simulink model "DiscretePIDTest"  (R2026b)
settings: Solver=FixedStepDiscrete  StopTime=pidTestCfg.Duration  FixedStep=pidCfg.Ts
PostLoadFcn:
  | addpath(fullfile(fileparts(get_param('DiscretePIDTest','FileName')),'..','build_process')); initialize_discrete_pid_test('DiscretePIDTest');
model workspace (MAT data in the model file):
  pidCfg.Kp = 1.2
  pidCfg.Ki = 8
  pidCfg.Kd = 0
  pidCfg.Tf = 0.01
  pidCfg.Ts = 0.001
  pidCfg.UMin = -1
  pidCfg.UMax = 1
  pidCfg.X0 = 0
  pidCfg.Kaw = 20
  pidCfg.PlantTau = 0.08
  pidCfg.ClosedLoop = 1
  pidStim.command.time = []
  pidStim.command.signals.values = [0 0 0 0 0 0 0 0 0 0 0 0 ... (3001 elements, 3001x1)]
  pidStim.command.signals.dimensions = 1
  pidStim.enable.time = []
  pidStim.enable.signals.values = [1 1 1 1 1 1 1 1 1 1 1 1 ... (3001 elements, 3001x1)]
  pidStim.enable.signals.dimensions = 1
  pidStim.reset.time = []
  pidStim.reset.signals.values = [0 0 0 0 0 0 0 0 0 0 0 0 ... (3001 elements, 3001x1)]
  pidStim.reset.signals.dimensions = 1
  pidTestCfg.Duration = 3
  pidTestCfg.CommandInitial = 0
  pidTestCfg.CommandHigh = 2
  pidTestCfg.CommandFinal = 0.2
  pidTestCfg.CommandTime = 0.1
  pidTestCfg.ReleaseTime = 1
  pidTestCfg.Enable = 1
  pidTestCfg.Reset = 0
libraries: slpidlib x1, DiscretePID x1
settings Model: Creator=24322  LastModifiedBy=24322
settings DataIOCC: SignalLogging=off

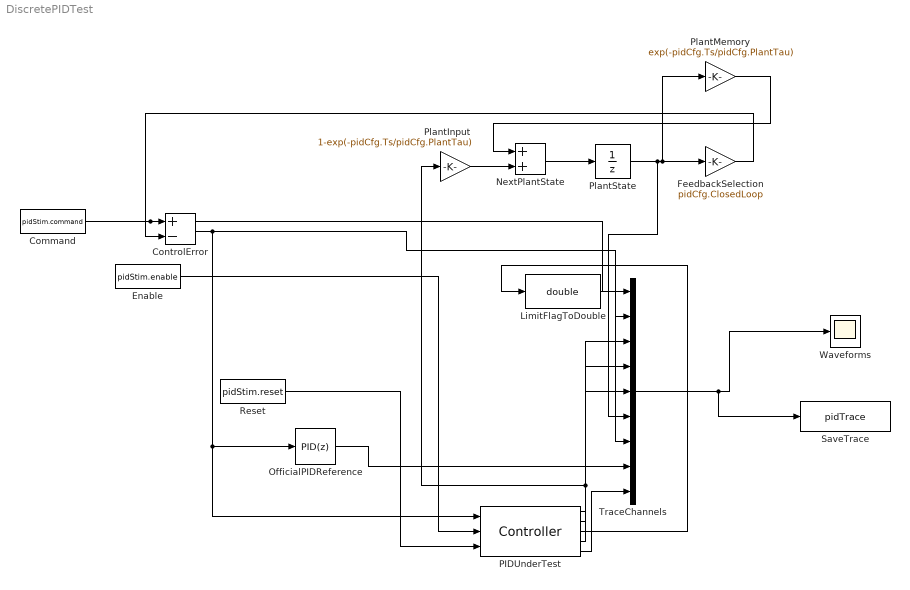
== system DiscretePIDTest ==
  Command : FromWorkspace  VariableName=pidStim.command  SampleTime=pidCfg.Ts  Interpolate=off  OutputAfterFinalValue=Holding final value
  ControlError : Sum  Inputs=+-
  Enable : FromWorkspace  VariableName=pidStim.enable  SampleTime=pidCfg.Ts  Interpolate=off  OutputAfterFinalValue=Holding final value
  FeedbackSelection : Gain  Gain=pidCfg.ClosedLoop
  LimitFlagToDouble : DataTypeConversion  OutDataTypeStr=double  SaturateOnIntegerOverflow=off  RndMeth=Floor
  NextPlantState : Sum
  OfficialPIDReference : slpidlib/PID Controller  Controller=PID  Form=Parallel  TimeDomain=Discrete-time  UseExternalTs=off  SampleTime=pidCfg.Ts  IntegratorMethod=Forward Euler  FilterMethod=Backward Euler  ControllerParametersSource=internal  P=pidCfg.Kp  I=pidCfg.Ki  UseKiTs=off  D=pidCfg.Kd  UseExternalDerivativeSource=off  N=1/pidCfg.Tf  UseFilter=on  TunerSelectOption=Transfer Function Based (PID Tuner App)  InitialConditionSource=internal  InitialConditionForIntegrator=pidCfg.X0  InitialConditionForFilter=0  DifferentiatorICPrevScaledInput=0  ExternalReset=none  TrackingMode=off  Kt=1  LimitOutput=on  SatLimitsSource=internal  UpperSaturationLimit=pidCfg.UMax  LowerSaturationLimit=pidCfg.UMin  LinearizeAsGain=off  AntiWindupMode=back-calculation  Kb=pidCfg.Kaw  LimitIntegrator=off  UpperIntegratorSaturationLimit=inf  LowerIntegratorSaturationLimit=-inf  POutMin=[]  POutMax=[]  IOutMin=[]  IOutMax=[]  DOutMin=[]  DOutMax=[]  NOutMin=[]  NOutMax=[]  SumOutMin=[]  SumOutMax=[]  SaturationOutMin=[]  SaturationOutMax=[]  PParamMin=[]  PParamMax=[]  IParamMin=[]  IParamMax=[]  DParamMin=[]  DParamMax=[]  NParamMin=[]  NParamMax=[]  KbParamMin=[]  KbParamMax=[]  KtParamMin=[]  KtParamMax=[]  KbOutMin=[]  KbOutMax=[]  KtOutMin=[]  KtOutMax=[]  IntegratorOutMin=[]  IntegratorOutMax=[]  FilterOutMin=[]  FilterOutMax=[]  SumI1OutMin=[]  SumI1OutMax=[]  SumI2OutMin=[]  SumI2OutMax=[]  SumI3OutMin=[]  SumI3OutMax=[]  SumI4OutMin=[]  SumI4OutMax=[]  SumDOutMin=[]  SumDOutMax=[]  DifferentiatorOutMin=[]  DifferentiatorOutMax=[]  FilterDiffOutCoefMin=[]  FilterDiffOutCoefMax=[]  ReciprocalOutMin=[]  ReciprocalOutMax=[]  SumDenOutMin=[]  SumDenOutMax=[]  SumNumOutMin=[]  SumNumOutMax=[]  DivideOutMin=[]  DivideOutMax=[]  UdiffTsProdOutMin=[]  UdiffTsProdOutMax=[]  NTsProdOutMin=[]  NTsProdOutMax=[]  UintegralTsProdOutMin=[]  UintegralTsProdOutMax=[]  UngainTsProdOutMin=[]  UngainTsProdOutMax=[]  ClampingZeroOutDataTypeStr=Inherit: Inherit via back propagation  ClampingZeroOutMin=[]  ClampingZeroOutMax=[]  FilterDenConstantOutDataTypeStr=Inherit: Inherit via back propagation  FilterDenConstantOutMin=[]  FilterDenConstantOutMax=[]  PCopyOutDataTypeStr=Inherit: Inherit via back propagation  PCopyOutMin=[]  PCopyOutMax=[]  NCopyOutDataTypeStr=Inherit: Inherit via back propagation  NCopyOutMin=[]  NCopyOutMax=[]  IntegratorContinuousStateAttributes=''  IntegratorStateMustResolveToSignalObject=off  IntegratorRTWStateStorageClass=Auto  FilterContinuousStateAttributes=''  FilterStateMustResolveToSignalObject=off  FilterRTWStateStorageClass=Auto  ParallelPVariant=InternalParameters  IdealPVariant=Disabled  IVariant=InternalParameters  DVariant=InternalParameters  IntegratorVariant=Discrete  SatVariant=Enabled  AWVariant=BackCalculation  PCopyVariant=Disabled  TRVariant=Disabled  FdbkBlocksVariant=Forward  IdealPFdbkVariant=Disabled  SatFdbkVariant=Disabled  DerivativeFilterVariant=BackwardEulerFilter  NVariant=InternalParameters  NCopyVariant=InternalParameters  FilterICVariant=InternalICsFilter  IntegratorICVariant=InternalICs  ExternalResetVariant=Disabled  TRSumVariant=Passthrough  SumFdbkVariant=Disabled  SumVariant=Sum_PID  TsampFilterVariant=InternalTs  TsampNgainVariant=Passthrough  TsampIntegralVariant=Disabled_SignalSpec  ExternalSaturationOutDataTypeStr=Inherit: Same as second input  DerivativeSourceVariant=ErrorSignal  PreIntVariant=InternalPreInt
      settings: LibrarySourceBlock=hdlsllib/Discrete/Discrete PID Controller
  PIDUnderTest : DiscretePID/Controller  Kp=pidCfg.Kp  Ki=pidCfg.Ki  Ts=pidCfg.Ts  UMin=pidCfg.UMin  UMax=pidCfg.UMax  X0=pidCfg.X0  Kaw=pidCfg.Kaw  Kd=pidCfg.Kd  Tf=pidCfg.Tf
  PlantInput : Gain  Gain=1-exp(-pidCfg.Ts/pidCfg.PlantTau)
  PlantMemory : Gain  Gain=exp(-pidCfg.Ts/pidCfg.PlantTau)
  PlantState : UnitDelay  SampleTime=pidCfg.Ts
  Reset : FromWorkspace  VariableName=pidStim.reset  SampleTime=pidCfg.Ts  Interpolate=off  OutputAfterFinalValue=Holding final value
  SaveTrace : ToWorkspace  VariableName=pidTrace  SaveFormat=Structure With Time  SampleTime=-1
  TraceChannels : Mux  Inputs=9
  Waveforms : Scope
      settings: ActiveDisplayYMinimum=-1  ActiveDisplayYMaximum=1
  wires:
  NextPlantState/1 -> PlantState/1
  PlantInput/1 -> NextPlantState/2
  PlantMemory/1 -> NextPlantState/1
  FeedbackSelection/1 -> ControlError/2
  PIDUnderTest/5 -> TraceChannels/9
  PIDUnderTest/4 -> TraceChannels/5
  PIDUnderTest/3 -> LimitFlagToDouble/1
  PIDUnderTest/2 -> TraceChannels/4
  PIDUnderTest/1 -> TraceChannels/3, PlantInput/1
  Reset/1 -> PIDUnderTest/3
  Enable/1 -> PIDUnderTest/2
  LimitFlagToDouble/1 -> TraceChannels/7
  ControlError/1 -> PIDUnderTest/1, OfficialPIDReference/1, TraceChannels/2
  Command/1 -> ControlError/1, TraceChannels/1
  PlantState/1 -> FeedbackSelection/1, PlantMemory/1, TraceChannels/6
  OfficialPIDReference/1 -> TraceChannels/8
  TraceChannels/1 -> SaveTrace/1, Waveforms/1
